simulink library "xps_library"  (Simulink 8.2)
settings: Solver=ode45  SolverMode=SingleTasking  StartTime=0.0  StopTime=10.0  RelTol=1e-3
undefined symbols (not defined in the file): sys_clk
libraries: xbsIndex_r4 x865, dspsigops x81, simulink x68, casper_library_flow_control x68, xps_library x25, casper_library_misc x4
(part 1 of 10)
settings Model: ForwardingTableString=||__slOldName__||xps_library/XSG core config||__slNewName__||xps_library/XSG_core_config||__slTransformationFcn__||XSG core config||__slOldName__||xps_library/Shared BRAM||__slNewName__||xps_library/Shared_BRAM||__slTransformationFcn__||Shared BRAM||__slOldName__||xps_library/software register||__slNewName__||xps_library/software_register||__slTransformationFcn__||Software Regsiter  Creator=hchen05  LastModifiedBy=jackh

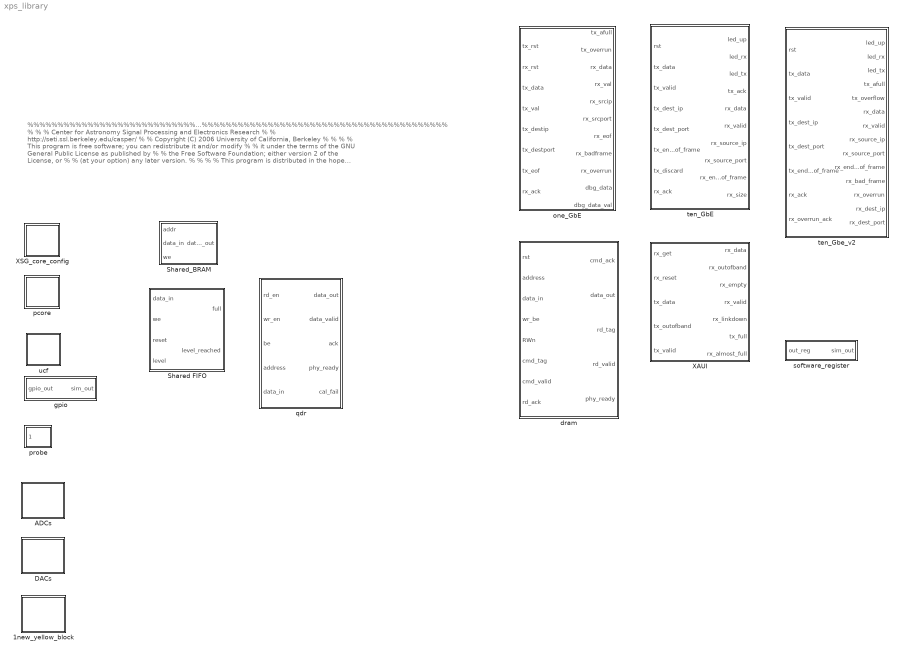
== system xps_library ==
  note: %%%%%%%%%%%%%%%%%%%%%%%%%%%%%%%%%%%%%%%%%%%%%%%%%%%%%%%%%%%%%%%%%%%%%%%%%%%%%%%
      | %                                                                             %
      | %   Center for Astronomy Signal Processing and Electronics Research           %
      | %   http://seti.ssl.berkeley.edu/casper/                                      %
      | %   Copyright (C) 2006 University of California, Berkeley                     %
      | %                                                                             %
      | %   This program is free software; you can redistribute it and/or modify      %
      | %   it under the terms of the GNU General Public License as published by      %
      | %   the Free Software Foundation; either version 2 of the License, or         %
      | %   (at your option) any later version.                                       %
      | %                                                                             %
      | %   This program is distributed in the hope that it will be useful,           %
      | %   but WITHOUT ANY WARRANTY; without even the implied warranty of            %
      | %   MERCHANTABILITY or FITNESS FOR A PARTICULAR PURPOSE.  See the             %
      | %   GNU General Public License for more details.                              %
      | %                                                                             %
      | %   You should have received a copy of the GNU General Public License along   %
      | %   with this program; if not, write to the Free Software Foundation, Inc.,   %
      | %   51 Franklin Street, Fifth Floor, Boston, MA 02110-1301 USA.               %
      | %                                                                             %
      | %%%%%%%%%%%%%%%%%%%%%%%%%%%%%%%%%%%%%%%%%%%%%%%%%%%%%%%%%%%%%%%%%%%%%%%%%%%%%%%
  1new_yellow_block : Subsystem  Tag=xps:block_name
  ADCs : Subsystem
  DACs : Subsystem
  Shared FIFO : Subsystem  Tag=xps:fifo  mask{io_dir=To Processor, arith_type=Unsigned, data_width=32, data_bin_pt=0, fifo_length=512}
      mask prompts: io_dir "I/O Direction:"; arith_type "Data Type:"; data_width "Data Width:"; data_bin_pt "Data Binary Point:"; fifo_length "Depth:"
      mask init:
      | fifo_mask;
      mask TypeOptions io_dir: From Processor | To Processor
      mask TypeOptions arith_type: Unsigned | Signed  (2's comp)
      mask TypeOptions data_width: 4 | 8 | 16 | 32 | 64 | 128 | 256
      mask TypeOptions fifo_length: 512 | 1024 | 2048 | 4096 | 8192 | 16384 | 32768 | 65536
  Shared_BRAM : Subsystem  Tag=xps:bram  mask{arith_type=Unsigned, addr_width=10, data_width=32, reg_prim_output=off, reg_core_output=off, optimization=Minimum_Area, data_bin_pt=0, init_vals=[0:2^10-1], sample_rate=1}
      mask prompts: arith_type "Output Data Type"; addr_width "Address width"; data_width "Data Width"; reg_prim_output "Register Primitive Output"; reg_core_output "Register Core Output"; data_bin_pt "Data Binary Point"; init_vals "Initial values (simulation only)"; sample_rate "Sample rate"
      mask init:
      | shared_bram_mask;
      mask TypeOptions arith_type: Unsigned | Signed  (2's comp)
      mask TypeOptions data_width: 8 | 16 | 32 | 64 | 128
      mask TypeOptions optimization: Minimum_Area | Low_Power
  XAUI : Subsystem  Tag=xps:xaui  mask(xaui){demux=1, port=ROACH:0, open_phy=on, show_param=off, pre_emph=3, swing=800}
      mask prompts: open_phy "Use KAT open PHY"; show_param "---------------------- Show Implementation Parameters -----------------------------------------------------------------------------------"; pre_emph "Pre-emphasis"; swing "Differential swing"
      mask help: XAUI block for sending and receiving point-to-point, streaming data over the ROACH1 CX4 connectors. NOTE: A new version of this block is in development.
      mask init:
      | xaui_mask;
      mask Help: eval('xlWeb([getenv(''MLIB_ROOT''), ''\doc\html\com_xaui\com_xaui.html''])')
      mask TypeOptions demux: 1 | 2
      mask TypeOptions port: ROACH:0 | ROACH:1 | ROACH:2 | ROACH:3
      mask Callback show_param:
      | myname=gcb;
      | if strcmp(get_param(myname, 'show_param'), 'on')
      |     set_param(myname, 'MaskVisibilities', {'on','on','on','on','on','on'});
      | else
      |     set_param(myname, 'MaskVisibilities', {'on','on','on','on','off','off'});
      | end
      mask TypeOptions pre_emph: 0 | 1 | 2 | 3
      mask TypeOptions swing: 400 | 500 | 600 | 700 | 800
  XSG_core_config : Subsystem  Tag=xps:xsg  mask(xsg core config){hw_sys=ROACH2:sx475t, clk_src=sys_clk, ROACH_clk_src=sys_clk, ROACH2_clk_src=sys_clk, MKDIG_clk_src=sys_clk, clk_rate=100, sample_period=1, synthesis_tool=XST}
      mask prompts: hw_sys "Hardware Platform"; clk_src "User IP Clock source"; ROACH_clk_src "User IP Clock Source"; ROACH2_clk_src "User IP Clock Source"; MKDIG_clk_src "User IP Clock Source"; clk_rate "User IP Clock Rate (MHz)"; sample_period "Sample Period"; synthesis_tool "Synthesis Tool:"
      mask help:
      | The XSG Core Config block is used to configure the System Generator design
      | for the casper_xps toolflow. Settings here are used to configure the
      | Xilinx System Generator block parameters automatically, and control toolflow
      | script  execution. It needs to be at the top level of all designs being compiled
      | with the casper_xps toolflow.
      mask init:
      | xps_xsg_conf_mask;
      mask Help: eval('xlWeb([getenv(''MLIB_ROOT''), ''\doc\html\sys_xsg_core_config\sys_xsg_core_config.html''])')
      mask TypeOptions hw_sys: ROACH:sx95t | ROACH:lx110t | ROACH2:sx475t | MKDIG
      mask Callback hw_sys: xps_xsg_conf_callback;
      mask TypeOptions ROACH_clk_src: sys_clk | sys_clk2x | arb_clk | aux0_clk | aux0_clk2x | aux1_clk | aux1_clk2x | adc0_clk | adc1_clk | dac0_clk | dac1_clk
      mask Callback ROACH_clk_src: xps_xsg_conf_callback;
      mask TypeOptions ROACH2_clk_src: sys_clk | aux_clk | adc0_clk | adc1_clk | dac0_clk | dac1_clk
      mask Callback ROACH2_clk_src: xps_xsg_conf_callback;
      mask TypeOptions MKDIG_clk_src: sys_clk | adc_clk
      mask Callback MKDIG_clk_src: xps_xsg_conf_callback;
      mask TypeOptions synthesis_tool: Leonardo Spectrum | Synplify | Synplify Pro | XST
      mask Display: fprintf(['MSSGE\n', hw_sys]);
  dram : Subsystem  Tag=xps:dram  mask(dram){dimm=1, arith_type=Unsigned, bin_pt=0, ip_clock=200, sample_period=1, bram_fifos=on, disable_tag=on, ram_depth=18, bank_mgt=off, wide_data=off, half_burst=off, use_sniffer=on}
      mask prompts: arith_type "Data Type"; bin_pt "Data binary point"; ip_clock "Datapath clock rate (MHz)"; sample_period "Sample period"; bram_fifos "Use BRAM FIFOs"; disable_tag "Disable tag FIFO"; ram_depth "Simulation address width"; bank_mgt "Enable bank management"; wide_data "Use wide data bus (288 bits)"; half_burst "Use half-burst"; use_sniffer "Include CPU Interface"
      mask help:
      | Interface to 1GB DDR2 DIMM of ROACH1 and the 2-4GB DDR3 DIMM of ROACH2.
      | Commands that are clocked-in are executed with an unknown delay, however, execution order is maintained.
      mask init:
      | dram_mask(gcb, wide_data);
      mask TypeOptions dimm: 1
      mask TypeOptions arith_type: Boolean | Unsigned | Signed  (2's comp)
      mask Callback wide_data:
      | myname=gcb;
      | if strcmp(get_param(myname, 'wide_data'), 'off')
      |     masks = get_param(myname, 'MaskEnables');
      |     masks{12} = 'on';
      |     set_param(myname, 'MaskEnables', masks);
      | else
      |     set_param(myname, 'half_burst', 'off');
      |     masks = get_param(myname, 'MaskEnables');
      |     masks{12} = 'off';
      |     set_param(myname, 'MaskEnables', masks);
      | end
  gpio : Subsystem  Tag=xps:gpio  mask(gpio){io_group=ROACH:aux0_clk, io_dir=out, arith_type=Boolean, bitwidth=1, bin_pt=0, bit_index=0, sample_period=1, use_single_ended=off, use_ddr=off, reg_iob=on, reg_clk_phase=0, termination=None}
      mask prompts: io_group "I/O group"; io_dir "I/O direction"; arith_type "Data Type"; bitwidth "Data bitwidth"; bin_pt "Data binary point"; bit_index "GPIO bit index"; sample_period "Sample period"; use_single_ended "Use as single-ended"; use_ddr "Use DDR"; reg_iob "Pack register in the pad"; reg_clk_phase "Register clock phase"; termination "Termination method"
      mask help: GPIO interfaces for ROACH and ROACH2 boards.
      mask init:
      | gpio_mask;
      mask TypeOptions io_group: ROACH:aux0_clk | ROACH:aux1_clk | ROACH:led | ROACH:gpioa | ROACH:gpioa_oe_n | ROACH:gpiob | ROACH:gpiob_oe_n | ROACH:qsh | ROACH:zdok0 | ROACH:zdok1 | ROACH2:aux_clk | ROACH2:led | ROACH2:gpio | ROACH2:qsh | ROACH2:sync_in | ROACH2:sync_out | ROACH2:zdok0 | ROACH2:zdok1
      mask Callback io_group:
      | if ~isempty(find(strcmp(get_param(gcb, 'io_group'), {'ROACH:qsh' 'ROACH:zdok0' 'ROACH:zdok1' 'ROACH2:sync_in' 'ROACH2:sync_out'})))
      |     set_param(gcb, 'MaskVisibilities', {'on','on','on','on','on','on','on','on','on','on','on','on'});
      | else
      |     set_param(gcb, 'MaskVisibilities', {'on','on','on','on','on','on','on','off','on','on','on','on'});
      | end
      mask TypeOptions io_dir: in | out
      mask Callback io_dir:
      | if ~isempty(find(strcmp(get_param(gcb, 'io_group'), {'ROACH:qsh' 'ROACH:zdok0' 'ROACH:zdok1' 'ROACH2:sync_in' 'ROACH2:sync_out'})))
      |     set_param(gcb, 'MaskVisibilities', {'on','on','on','on','on','on','on','on','on','on','on','on'});
      | else
      |     set_param(gcb, 'MaskVisibilities', {'on','on','on','on','on','on','on','off','on','on','on','on'});
      | end
      mask TypeOptions arith_type: Boolean | Unsigned | Signed  (2's comp)
      mask Callback use_ddr:
      | if strcmp(get_param(gcb,'use_ddr'),'on')
      |     set_param(gcb,'reg_iob','on');
      |     set_param(gcb,'MaskEnables', {'on' 'on' 'on' 'on' 'on' 'on' 'on' 'on' 'on' 'off' 'on' 'on'});
      | else
      |     set_param(gcb,'MaskEnables', {'on' 'on' 'on' 'on' 'on' 'on' 'on' 'on' 'on' 'on' 'on' 'on'});
      | end
      mask TypeOptions reg_clk_phase: 0 | 90 | 180 | 270
      mask TypeOptions termination: None | Pullup | Pulldown
  one_GbE : Subsystem  Tag=xps:onegbe  mask(one_GbE){local_en=on, dis_cpu_rx=off, dis_cpu_tx=off, cpu_promiscuous=on, local_mac=hex2dec('123456789abc'), local_ip=hex2dec('c0a8290a'), local_port=4321, local_gateway=1}
      mask prompts: local_en "Enable fabric on startup"; dis_cpu_rx "Disable CPU Rx"; dis_cpu_tx "Disable CPU Tx"; cpu_promiscuous "CPU Promiscuous"; local_mac "Fabric MAC Address"; local_ip "Fabric IP Address"; local_port "Fabric UDP Port"; local_gateway "Fabric Gateway"
      mask help: This block sends and receives UDP frames (packets). It accepts a 8 bit wide data stream with user-determined frame breaks. The data stream is wrapped in a UDP frame for transmission. Incoming UDP packets are unwrapped and the data presented as a 8 bit wide stream.
      mask init:
      | onegbe_mask;
      mask Help: eval('xlWeb([getenv(''MLIB_ROOT''), ''\doc\html\com_ten_GbE\com_ten_GbE.html''])')
  pcore : Subsystem  Tag=xps:pcore  mask(pcore){pcore_path=customlib/pcores}
      mask prompts: pcore_path "Custom pcores path"
      mask help: Allows insertion of custom EDK pcores not distributed with base systems.
      mask Display: fprintf('PCORE');
  probe : Subsystem  Tag=xps:probe  mask{ila_number=0, match_type=basic, match_counter_width=8, capture_depth=512, arith_type=Boolean, bitwidth=1, bin_pt=0}
      mask prompts: ila_number "Chipscope ILA number"; match_type "Match Unit Type"; match_counter_width "Match counter width"; capture_depth "Probe capture depth"; arith_type "Data type"; bitwidth "Data bit width"; bin_pt "Data binary point"
      mask init:
      | probe_mask;
      mask TypeOptions ila_number: 0 | 1 | 2 | 3 | 4 | 5 | 6 | 7 | 8 | 9 | 10 | 11 | 12 | 13 | 14
      mask TypeOptions match_type: basic | basic with edges | extended | extended with edges | range | range with edges
      mask TypeOptions match_counter_width: 0 | 8 | 16 | 24 | 32
      mask TypeOptions capture_depth: 512 | 1024 | 2048 | 4096 | 8192 | 16384
      mask TypeOptions arith_type: Boolean | Unsigned | Signed  (2's comp)
  qdr : Subsystem  Tag=xps:qdr  mask(qdr){which_qdr=qdr0, qdr_awidth=12, use_sniffer=on}
      mask prompts: which_qdr "QDR Chip"; qdr_awidth "Simulation QDR address width"; use_sniffer "Include CPU Interface"
      mask help:
      | Interface to the QDR II SRAM device on ROACH and ROACH2.
      | For ROACH, use only QDR chips qdr0 or qdr1.
      | For ROACH2, use qdr chips qdr0, qdr1, qdr2 or qdr3.
      mask init:
      | qdr_mask(gcb);
      mask TypeOptions which_qdr: qdr0 | qdr1 | qdr2 | qdr3
  software_register : Subsystem  Tag=xps:sw_reg  mask(swreg){io_dir=To Processor, io_delay=0, sample_period=1, names=reg, bitwidths=32, bin_pts=0, arith_types=0, sim_port=on, show_format=on}
      mask prompts: io_dir "I/O direction"; io_delay "I/O delay"; sample_period "Sample period"; names "Bitfield names [msb...lsb]"; bitwidths "Bitfield widths"; bin_pts "Bitfield binary pts"; arith_types "Bitfield types, ufix=0, fix=1, bool=2"; sim_port "Provide sim input/output?"; show_format "Print format string?"
      mask help: A 32-bit software-accessible register. Can be divided into bitfields of varying widths and types using the fields in the block mask.
      mask init:
      | try
      |     swreg_init(gcb)
      | catch ex
      |     disp(sprintf('%s: %s', gcb, ex.message))
      |     errordlg(ex.message)
      | end
      settings: AttributesFormatString=1output:uf32.0 = 32 bits
      mask TypeOptions io_dir: To Processor | From Processor
      mask Callback io_dir:
      | mask_enables = get_param(gcb, 'MaskEnables');
      | mask_names = get_param(gcb, 'MaskNames');
      | if strcmp(get_param(gcb, 'io_dir'), 'To Processor'),
      |     mask_enables{ismember(mask_names, 'sample_period')} = 'off';
      | else
      |     mask_enables{ismember(mask_names, 'sample_period')} = 'on';
      | end
      | set_param(gcb, 'MaskEnables', mask_enables);
  ten_GbE : Subsystem  Tag=xps:tengbe  mask(ten_GbE){port=ROACH:0, mac_lite=off, open_phy=off, show_param=off, pre_emph=3, swing=800, fab_en=off, fab_mac=0, fab_ip=0, fab_udp=0, fab_gate=0}
      mask prompts: mac_lite "Use light-weight MAC: Warning --> it DOES NOT check any CRC on receive"; open_phy "Use KAT open XAUI PHY"; show_param "---------------------- Show Implementation Parameters -----------------------------------------------------------------------------------"; pre_emph "Pre-emphasis"; swing "Differential swing"; fab_en "Enable fabric on startup"; fab_mac "Fabric MAC Address"; fab_ip "Fabric IP Address"; fab_udp "Fabric UDP Port"; fab_gate "Fabric Gateway"
      mask help: This block sends and receives UDP frames (packets). It accepts a 64 bit wide data stream with user-determined frame breaks. The data stream is wrapped in a UDP frame for transmission. Incoming UDP packets are unwrapped and the data presented as a 64 bit wide stream.
      mask init:
      | tengbe_mask;
      mask Help: eval('xlWeb([getenv(''MLIB_ROOT''), ''\doc\html\com_ten_GbE\com_ten_GbE.html''])')
      mask TypeOptions port: ROACH:0 | ROACH:1 | ROACH:2 | ROACH:3
      mask Callback show_param:
      | myname=gcb;
      | if strcmp(get_param(myname, 'show_param'), 'on')
      |     set_param(myname, 'MaskVisibilities', {'on','on','on','on','on', 'on','on','on','on','on', 'on',});
      | else
      |     set_param(myname, 'MaskVisibilities', {'on','on','on','on','off','off','off','off','off','off','off'});
      | end
      mask TypeOptions pre_emph: 0 | 1 | 2 | 3
      mask TypeOptions swing: 400 | 500 | 600 | 700 | 800
  ten_Gbe_v2 : Subsystem  Tag=xps:tengbe_v2  mask(ten_GbE_v2){flavour=sfp+, slot=0, port_r1=0, port_r2_cx4=0, port_r2_sfpp=0, rx_dist_ram=off, large_frames=off, show_param=off, pre_emph_r2=1.07, pre_emph=3, post_emph_r2=0.18, rxeqmix_r2=7, swing_r2=940, swing=800, fab_en=on, fab_mac=hex2dec('123456780000'), fab_ip=192*(2^24) + 168*(2^16) + 5*(2^8) + 20*(2^0), fab_udp=10000, fab_gate=1, cpu_rx_en=on, cpu_tx_en=on, ttl=hex2dec('FF'), promisc_mode=off, debug_ctr_width=16, txctr=off, txerrctr=off, txerrctr_len=100, txofctr=off, txfullctr=off, txvldctr=off, txsnaplen=0 - no snap, rxctr=off, rxerrctr=off, rxerrctr_len=100, rxofctr=off, rxbadctr=off, rxvldctr=off, rxeofctr=off, rxsnaplen=0 - no snap}
      mask prompts: flavour "Mezzanine card flavour"; slot "Card slot"; port_r1 "Port"; port_r2_cx4 "Port"; port_r2_sfpp "Port"; rx_dist_ram "Shallow RX Fifo (Beware overruns!)"; large_frames "Enable Large TX Frames (8k+512)"; show_param "---------------------- Show Implementation Parameters -----------------------------------------------------------------------------------"; pre_emph_r2 "Pre-emphasis (dB)"; pre_emph "Pre-emphasis"; post_emph_r2 "Post-emphasis (dB)"; rxeqmix_r2 "Receive equalisation"; swing_r2 "Driver Swing Control (mVppd)"; swing "Differential swing"; fab_en "Enable fabric on startup"; fab_mac "Fabric MAC Address"; fab_ip "Fabric IP Address"; fab_udp "Fabric UDP Port"; fab_gate "Fabric Gateway"; cpu_rx_en "Enable CPU RX"; cpu_tx_en "Enable CPU TX"; promisc_mode "Promiscuous mode"; debug_ctr_width "Debug counter width"; txctr "TX - core_txctr"; txerrctr "TX packet length error - core_txerrctr"; txerrctr_len "-- expected TX packet length"; txofctr "TX overflow - core_txofctr"; txfullctr "TX full - core_txfullctr"; txvldctr "TX valid cycle - core_txvldctr"; txsnaplen "TX snapshot length"; rxctr "RX - core_rxctr"; rxerrctr "RX packet length error - core_rxerrctr"; rxerrctr_len "-- expected RX packet length"; rxofctr "RX overflow - core_rxofctr"; rxbadctr "RX bad - core_rxbadctr"; rxvldctr "RX valid cycle - core_rxvldctr"; rxeofctr "RX eof - core_rxeofctr"; rxsnaplen "RX snapshot length"
      mask help: This block sends and receives UDP frames (packets). It accepts a 64 bit wide data stream with user-determined frame breaks. The data stream is wrapped in a UDP frame for transmission. Incoming UDP packets are unwrapped and the data presented as a 64 bit wide stream.
      mask init:
      | temp = eval(get_param(gcb, 'debug_ctr_width'));
      | if temp <= 0,
      |     error('Debug counters cannot be ltoet zero.');
      | end
      | tengbe_v2_mask(gcb)
      mask TypeOptions flavour: sfp+ | cx4
      mask Callback flavour: tengbe_v2_callback
      mask TypeOptions slot: 0 | 1
      mask TypeOptions port_r1: 0 | 1 | 2 | 3
      mask TypeOptions port_r2_cx4: 0 | 1 | 2
      mask TypeOptions port_r2_sfpp: 0 | 1 | 2 | 3
      mask Callback show_param: tengbe_v2_callback
      mask TypeOptions pre_emph_r2: 0.15 | 0.3 | 0.45 | 0.61 | 0.74 | 0.91 | 1.07 | 1.25 | 1.36 | 1.55 | 1.74 | 1.94 | 2.11 | 2.32 | 2.54 | 2.77
      mask TypeOptions pre_emph: 0 | 1 | 2 | 3
      mask TypeOptions post_emph_r2: 0.18 | 0.19 | 0.2 | 0.39 | 0.63 | 0.82 | 1.07 | 1.32 | 1.6 | 1.65 | 1.94 | 2.21 | 2.52 | 2.76 | 3.08 | 3.41 | 3.77 | 3.97 | 4.36 | 4.73 | 5.16 | 5.47 | 5.93 | 6.38 | 6.89
      mask TypeOptions rxeqmix_r2: 0 | 1 | 2 | 3 | 4 | 5 | 6 | 7
      mask TypeOptions swing_r2: 110 | 210 | 310 | 400 | 480 | 570 | 660 | 740 | 810 | 880 | 940 | 990 | 1040 | 1080 | 1110 | 1130
      mask TypeOptions swing: 400 | 500 | 600 | 700 | 800
      mask Callback txerrctr:
      | blk = gcb;
      | mask_visibilities = get_param(blk, 'MaskVisibilities');
      | mask_names = get_param(blk, 'MaskNames');
      | if strcmp(get_param(blk, 'txerrctr'), 'on')
      |     mask_visibilities{ismember(mask_names, 'txerrctr_len')} = 'on';
      | else
      |     mask_visibilities{ismember(mask_names, 'txerrctr_len')} = 'off';
      | end
      | set_param(blk, 'MaskVisibilities', mask_visibilities);
      mask TypeOptions txsnaplen: 0 - no snap | 256 | 512 | 1024 | 2048 | 4096 | 8192 | 16384
      mask Callback rxerrctr:
      | blk = gcb;
      | mask_visibilities = get_param(blk, 'MaskVisibilities');
      | mask_names = get_param(blk, 'MaskNames');
      | if strcmp(get_param(blk, 'rxerrctr'), 'on')
      |     mask_visibilities{ismember(mask_names, 'rxerrctr_len')} = 'on';
      | else
      |     mask_visibilities{ismember(mask_names, 'rxerrctr_len')} = 'off';
      | end
      | set_param(blk, 'MaskVisibilities', mask_visibilities);
      mask TypeOptions rxsnaplen: 0 - no snap | 256 | 512 | 1024 | 2048 | 4096 | 8192 | 16384
  ucf : Subsystem  Tag=xps:ucf  mask(ucf){ucf_file=/tmp/testucf.ucf}
      mask prompts: ucf_file "Path to file containing constraints. (This should adhere to .ucf syntax)"
      mask help: Allows insertion of custom constraints into a compile.
      mask Display: fprintf('UCF');

== system xps_library/1new_yellow_block ==

== system xps_library/ADCs ==
  adc : Subsystem  Tag=xps:adc  mask(adc){adc_brd=adc0, adc_clk_rate=800, adc_interleave=on, sample_period=1}
      mask prompts: adc_brd "ADC board"; adc_clk_rate "ADC clock rate (MHz)"; adc_interleave "ADC interleave mode"; sample_period "Sample period"
      mask help: The ADC block converts analog inputs to digital outputs. Every clock cycle, the inputs are sampled and digitized to 8 bit binary point numbers in the range of [-1, 1) and are then output by the adc.
      mask init:
      | adc_mask;
      mask Help: eval('xlWeb([getenv(''MLIB_ROOT''), ''\doc\html\sys_adc\sys_adc.html''])')
      mask TypeOptions adc_brd: adc0 | adc1
  adc083000_ctrl : Subsystem  Tag=xps:adc083000_ctrl  mask(adc083000_ctrl){}
      mask init:
      | adc083000_ctrl_mask;
  adc083000x2 : Subsystem  Tag=xps:adc083000x2  mask(adc_083000x2){use_adc0=on, use_adc1=on, demux_adc=off, clock_sync=on, verbose=off, using_ctrl=on, adc_clk_rate=1000, sample_period=1, bit_width=8}
      mask prompts: use_adc0 "Use ZD0K0?"; use_adc1 "Use ZDOK1?"; demux_adc "Demux ADCs by 2?"; clock_sync "Interleave 2 ADC boards?"; verbose "Verbose Block Creation?"; using_ctrl "Add ports for control registers?"; adc_clk_rate "ADC clock rate (MHz)"; sample_period "Sample Period"; bit_width "Output Bit Width"
      mask help:
      | The ADC block converts analog inputs to digital outputs.
      | Every clock cycle, the inputs are sampled and digitized to
      | 8 bit binary point numbers in the range of [-1, 1).
      |
      | Online block-specific documentation: http://casper.berkeley.edu/wiki/Adc083000
      mask init:
      | adc083000_mask;
      mask Help: eval('xlWeb([getenv(''MLIB_ROOT''), ''\doc\html\sys_adc\sys_adc.html''])')
  adc16x250-8 : Subsystem  Tag=xps:adc16  mask(ADC16){board_count=1, roach2_rev=2, zdok_rev=2}
      mask prompts: board_count "Number of ADC16 Boards"; roach2_rev "ROACH2 Revision"; zdok_rev "ZDOK Pinout Revision"
      mask help: 16-input ADC. When using one ADC16 board, it must be in ZDOK0.
      mask init:
      | % Only board_count is needed by init function
      | adc16_init(gcb, ...
      |     'board_count', board_count);
      settings: AttributesFormatString=r2 rev%<roach2_rev>\nzdok rev%<zdok_rev>
      mask Help:
      | This is the CASPER "yellow block" for the CASPER ADC16 board.  Each ADC
      | board has four ADC chips.  Each ADC chip accepts four inputs.  The four
      | 8-bit outputs from each ADC chip are concatenated into a 32-bit signal.
      mask TypeOptions board_count: 1 | 2
      mask TypeOptions roach2_rev: 1 | 2
      mask TypeOptions zdok_rev: 1 | 2
  adc1x1800-10 : Subsystem  Tag=xps:mkadc  mask(mkadc){adc_brd=adc0, adc_clk_rate=1800, sample_period=1, gray_en=on}
      mask prompts: adc_brd "ADC board"; adc_clk_rate "ADC clock rate (MHz)"; sample_period "Sample period"; gray_en "Gray Code Enable"
      mask help:
      | ADC1x1800-10
      | Single Input, Max 1.8G Sample, 10bit
      | Demux by 4
      | ADC: e2v AT84AS008CGL
      | DEMUX by 2: AT84CS001VTP
      | DEMUX by 2: FPGA
      mask init:
      | mkadc_mask;
      mask Help: ADC1x1800
      mask TypeOptions adc_brd: adc0 | adc1
  adc2x14_400 : Subsystem  Tag=xps:adc2x14_400  mask(ADC board 2xADS5474 Interface Block){adc_brd=0, adc_clk_rate=400}
      mask prompts: adc_brd "ADC Board"; adc_clk_rate "ADC Clock Rate (MHz)"
      mask help: Interface block for the MKID 14-bits 400 MHz ADC board (2xADS5474).
      mask init:
      | adc2x14_400_mask;
      mask TypeOptions adc_brd: 0 | 1
  adc2x14_400_4x : Subsystem  Tag=xps:adc2x14_400_4x  mask(2x 14-400 ADC Interface Block){adc_brd=1, adc_clk_rate=400}
      mask prompts: adc_brd "ADC Board"; adc_clk_rate "ADC Clock Rate (MHz)"
      mask help: Interface block for the 14-bits 400 MHz DC board (2xADS5474).
      mask init:
      | adc2x14_400_4x_mask;
      mask TypeOptions adc_brd: 0 | 1
  adc_mkid : Subsystem  Tag=xps:adc_mkid  mask(MKID ADC Interface Block){adc_brd=1, adc_clk_rate=512}
      mask prompts: adc_brd "ADC Board"; adc_clk_rate "ADC Clock Rate (MHz)"
      mask help: Interface block for the MKID 12-bits 550 MHz ADC board (2xADS54RF63).
      mask init:
      | adc_mkid_mask;
      mask TypeOptions adc_brd: 0 | 1
  adc_mkid_4x : Subsystem  Tag=xps:adc_mkid_4x  mask(MKID ADC Interface Block){adc_brd=1, adc_clk_rate=540}
      mask prompts: adc_brd "ADC Board"; adc_clk_rate "ADC Clock Rate (MHz)"
      mask help: Interface block for the MKID 12-bits ADC board (2xADS54RF63).
      mask init:
      | adc_mkid_4x_mask;
      mask TypeOptions adc_brd: 0 | 1
  adc_sim : Subsystem  mask(adc_sim){nStreams=8, bit_width=8}
      mask prompts: nStreams "Number of Output Streams"; bit_width "Sample Bit Width"
      mask help:
      | This block simulates the behavior of a demuxed ADC, which takes
      | as input a waveform and returns digital samples in parallel at
      | a slower rate.
      |
      | This block is used to simulate the behavior
      mask init:
      | adc_sim_init(gcb, ...
      |     'nStreams', nStreams, ...
      |     'bit_width', bit_width);
  asiaa_adc5g : Subsystem  Tag=xps:adc5g  mask(adc5g){input_mode=One-channel -- A, adc_brd=ZDOK 0, demux=1:2, adc_bit_width=4, adc_clk_rate=2500, using_ctrl=on, test_ramp=off}
      mask prompts: input_mode "Input mode:"; adc_brd "ADC Board"; demux "Internal demux"; adc_bit_width "ADC Resolution (bits):"; adc_clk_rate "ADC Clock Rate (MHz):"; using_ctrl "use control"; test_ramp "start in test ramp mode"
      mask help:
      | Interface for the ASIAA 5 GSps ADC. Supports interleaving all four
      | cores using either input A or C, or interleaving two-cores each for
      | A and C. The hardware itself comes in two versions:
      |
      | DMUX 1:2 -- 4-bit samples, 4 parallel streams
      | DMUX 1:1 -- 8-bit samples, 2 parallel streams
      |
      | In either configuration this block will output 8 parallel streams
      | but the underlying interface, and the bitwidth of the samples,
      | will be different.
      mask init:
      | adc5g_init(gcb,...
      |     'input_mode', input_mode,...
      |     'demux', demux,...
      |     'adc_clk_rate', adc_clk_rate,...
      |     'adc_bit_width', adc_bit_width,...
      |     'adc_brd', adc_brd,...
      |     'using_ctrl', using_ctrl,...
      |     'test_ramp', test_ramp);
      mask TypeOptions input_mode: One-channel -- A | One-channel -- C | Two-channel -- A&C
      mask TypeOptions adc_brd: ZDOK 0 | ZDOK 1
      mask TypeOptions demux: 1:1 | 1:2
      mask Callback demux:
      | demux = get_param(gcb,'demux');
      | if(strcmp(demux,'1:1')),
      |     set_param(gcb, 'adc_bit_width', '8')
      | elseif(strcmp(demux, '1:2')),
      |     set_param(gcb, 'adc_bit_width', '4');
      | else
      | end
  conv : Subsystem  mask{bit_width=8}
      mask prompts: bit_width "Bit Width"
      mask help:
      | Converts an (8-bit) unsigned number to 2's complement.
      | This block should eventually be able to handle arbitrary
      | width inputs.
      mask init:
      | % set_param([gcb, '/Slice1'], 'nbits', num2str(bit_width-1));
      | % set_param([gcb, '/Reinterpret'], 'bin_pt', num2str(bit_width-1));
  generic_adc : Subsystem  mask(generic_adc){in=1, out=4, bits=8, interleaved=off, or_support=off, sync_support=on, dv_support=off}
      mask prompts: in "inputs"; out "outputs per input"; bits "adc bit width"; interleaved "interleaved mode"; or_support "over-range support"; sync_support "sync support"; dv_support "data valid support"
      mask help: Generic ADC simulation block
      mask init:
      | generic_adc_init(gcb, ...
      |     'in', in, ...
      |     'out', out, ...
      |     'bits', bits, ...    
      |     'interleaved', interleaved, ...
      |     'or_support', or_support, ...
      |     'sync_support', sync_support, ...
      |     'dv_support', dv_support);
  katadc : Subsystem  Tag=xps:katadc  mask(katadc){adc_brd=adc0, adc_interleave=off, bypass_auto=off, en_gain=on, adc_clk_rate=800, sample_period=1}
      mask prompts: adc_brd "ADC board"; adc_interleave "ADC interleave mode"; bypass_auto "Bypass auto config"; en_gain "Enable gain"; adc_clk_rate "ADC sampling rate (MHz)"; sample_period "Sample period"
      mask init:
      | name = gcb;
      | katadc_init(gcb, ...
      |     'name', name, ...
      |     'adc_brd', adc_brd, ...
      |     'adc_interleave', adc_interleave, ...
      |     'bypass_auto', bypass_auto, ...
      |     'en_gain', en_gain, ...
      |     'adc_clk_rate', adc_clk_rate, ...
      |     'sample_period', sample_period);
      mask TypeOptions adc_brd: adc0 | adc1
  of1 : Subsystem  mask(of){bit_num=0, n_adc_bits=8}
      mask prompts: bit_num "Bit index of overflow detection bus:"; n_adc_bits "Number of bits in ADC"
      mask help: 1-cycle overflow detector for an n-bit ADC outputs (simulation only)
  of_detect_bus : Subsystem  mask(of_detect_bus){nStreams=8, bit_width=8}
      mask prompts: nStreams "Number of Streams"; bit_width "Bit Width"
      mask init:
      | of_detect_bus_init(gcb, ...
      |     'nStreams', nStreams, ...
      |     'bit_width', bit_width);
  quadc : Subsystem  Tag=xps:quadc  mask(CASPER QuADC Interface Block){adc_brd=0, adc_clk_rate=200}
      mask prompts: adc_brd "ADC Board"; adc_clk_rate "ADC Clock Rate (MHz)"
      mask help: Interface block for the CASPER Quad ADC board (ADC4x250-8).
      mask init:
      | quadc_mask;
      mask TypeOptions adc_brd: 0 | 1
  x64_adc : Subsystem  Tag=xps:x64_adc  mask(x64_adc){adc_clk_rate=12, spi=off, ctrl_gpio=GPIO_A}
      mask prompts: adc_clk_rate "ADC clock rate (MHz)"; spi "Include SPI interface?"; ctrl_gpio "GPIO bank to use for control signals?"
      mask help: The ADC block converts analog inputs to digital outputs. Every clock cycle, the inputs are sampled and digitized to 8 bit binary point numbers in the range of [-1, 1) and are then output by the adc.
      mask init:
      | x64_adc_mask(gcb, 'spi', spi);
      mask Help: eval('xlWeb([getenv(''MLIB_ROOT''), ''\doc\html\sys_adc\sys_adc.html''])')
      mask TypeOptions ctrl_gpio: GPIO_A | GPIO_B

== system xps_library/DACs ==
  dac_mkid : Subsystem  Tag=xps:dac_mkid  mask(MKID DAC Interface Block){dac_brd=0, dac_clk_rate=512, sample_period=1}
      mask prompts: dac_brd "DAC board"; dac_clk_rate "DAC external clock rate (MHz)"; sample_period "Sample period"
      mask help: Interface block for the MKID 16-bits DAC board (2xDAC5681)
      mask init:
      | dac_mkid_mask;
      mask TypeOptions dac_brd: 0 | 1
  dac_mkid_4x : Subsystem  Tag=xps:dac_mkid_4x  mask{dac_brd=0, dac_clk_rate=540, sample_period=1}
      mask prompts: dac_brd "DAC board"; dac_clk_rate "DAC external clock rate (MHz)"; sample_period "Sample period"
      mask init:
      | dac_mkid_4x_mask;
      mask TypeOptions dac_brd: 0 | 1

== system xps_library/Shared FIFO ==
  data_in : Inport
  we : Inport  Port=2
  reset : Inport  Port=3
  level : Inport  Port=4
  convert_untitled_Shared_FIFO_user_data_in : xbsIndex_r4/Convert  gui_display_data_type=Fixed-point  arith_type=Unsigned  n_bits=32  bin_pt=0  float_type=Single  exp_bits=8  fraction_bits=24  quantization=Truncate  overflow=Wrap  en=off  latency=0  dbl_ovrd=off  pipeline=off  block_type=convert
  convert_untitled_Shared_FIFO_user_level : xbsIndex_r4/Convert  gui_display_data_type=Fixed-point  arith_type=Unsigned  n_bits=16  bin_pt=0  float_type=Single  exp_bits=8  fraction_bits=24  quantization=Truncate  overflow=Wrap  en=off  latency=0  dbl_ovrd=off  pipeline=off  block_type=convert
  convert_untitled_Shared_FIFO_user_reset : xbsIndex_r4/Convert  gui_display_data_type=Fixed-point  arith_type=Unsigned  n_bits=1  bin_pt=0  float_type=Single  exp_bits=8  fraction_bits=24  quantization=Truncate  overflow=Wrap  en=off  latency=0  dbl_ovrd=off  pipeline=off  block_type=convert
  convert_untitled_Shared_FIFO_user_we : xbsIndex_r4/Convert  gui_display_data_type=Fixed-point  arith_type=Unsigned  n_bits=1  bin_pt=0  float_type=Single  exp_bits=8  fraction_bits=24  quantization=Truncate  overflow=Wrap  en=off  latency=0  dbl_ovrd=off  pipeline=off  block_type=convert
  untitled_Shared_FIFO_user_data_in : xbsIndex_r4/Gateway Out  hdl_port=on  timing_constraint=None  locs_specified=off  LOCs={}  block_type=gatewayout
      settings: infoedit="Gateway out block.  Converts Xilinx fixed point inputs into ouputs of type Simulink integer, double, or fixed point.<P><P>Hardware notes:  In hardware these blocks become top level output ports or are discarded, depending on how they are configured."
  untitled_Shared_FIFO_user_full : xbsIndex_r4/Gateway In  gui_display_data_type=Fixed-point  arith_type=Unsigned  n_bits=1  bin_pt=0  preci_type=Single  exp_width=8  frac_width=24  quantization="Round  (unbiased: +/- Inf)"  overflow=Saturate  period=1  dbl_ovrd=off  timing_constraint=None  locs_specified=off  LOCs={}  hdl_port=on  block_type=gatewayin
      settings: infoedit="Gateway in block.  Converts inputs of type Simulink integer, double and fixed point to  Xilinx fixed point type.<P><P>Hardware notes:  In hardware these blocks become top level input ports."
  untitled_Shared_FIFO_user_full_const : Constant  Value=0
  untitled_Shared_FIFO_user_level : xbsIndex_r4/Gateway Out  hdl_port=on  timing_constraint=None  locs_specified=off  LOCs={}  block_type=gatewayout
      settings: infoedit="Gateway out block.  Converts Xilinx fixed point inputs into ouputs of type Simulink integer, double, or fixed point.<P><P>Hardware notes:  In hardware these blocks become top level output ports or are discarded, depending on how they are configured."
  untitled_Shared_FIFO_user_level_reached : xbsIndex_r4/Gateway In  gui_display_data_type=Fixed-point  arith_type=Unsigned  n_bits=1  bin_pt=0  preci_type=Single  exp_width=8  frac_width=24  quantization="Round  (unbiased: +/- Inf)"  overflow=Saturate  period=1  dbl_ovrd=off  timing_constraint=None  locs_specified=off  LOCs={}  hdl_port=on  block_type=gatewayin
      settings: infoedit="Gateway in block.  Converts inputs of type Simulink integer, double and fixed point to  Xilinx fixed point type.<P><P>Hardware notes:  In hardware these blocks become top level input ports."
  untitled_Shared_FIFO_user_level_reached_const : Constant  Value=0
  untitled_Shared_FIFO_user_reset : xbsIndex_r4/Gateway Out  hdl_port=on  timing_constraint=None  locs_specified=off  LOCs={}  block_type=gatewayout
      settings: infoedit="Gateway out block.  Converts Xilinx fixed point inputs into ouputs of type Simulink integer, double, or fixed point.<P><P>Hardware notes:  In hardware these blocks become top level output ports or are discarded, depending on how they are configured."
  untitled_Shared_FIFO_user_we : xbsIndex_r4/Gateway Out  hdl_port=on  timing_constraint=None  locs_specified=off  LOCs={}  block_type=gatewayout
      settings: infoedit="Gateway out block.  Converts Xilinx fixed point inputs into ouputs of type Simulink integer, double, or fixed point.<P><P>Hardware notes:  In hardware these blocks become top level output ports or are discarded, depending on how they are configured."
  full : Outport
  level_reached : Outport  Port=2
  wires:
  untitled_Shared_FIFO_user_level_reached_const/1 -> untitled_Shared_FIFO_user_level_reached/1
  untitled_Shared_FIFO_user_level_reached/1 -> level_reached/1
  untitled_Shared_FIFO_user_full_const/1 -> untitled_Shared_FIFO_user_full/1
  untitled_Shared_FIFO_user_full/1 -> full/1
  convert_untitled_Shared_FIFO_user_level/1 -> untitled_Shared_FIFO_user_level/1
  level/1 -> convert_untitled_Shared_FIFO_user_level/1
  convert_untitled_Shared_FIFO_user_reset/1 -> untitled_Shared_FIFO_user_reset/1
  reset/1 -> convert_untitled_Shared_FIFO_user_reset/1
  convert_untitled_Shared_FIFO_user_we/1 -> untitled_Shared_FIFO_user_we/1
  we/1 -> convert_untitled_Shared_FIFO_user_we/1
  convert_untitled_Shared_FIFO_user_data_in/1 -> untitled_Shared_FIFO_user_data_in/1
  data_in/1 -> convert_untitled_Shared_FIFO_user_data_in/1

== system xps_library/Shared_BRAM ==
  addr : Inport
  data_in : Inport  Port=2
  we : Inport  Port=3
  calc_add : Subsystem  mask{data_width=32, addr_width=10, sample_rate=sample_rate}
      mask prompts: data_width "data width"; addr_width "address width"; sample_rate "sample rate"
  convert_addr : xbsIndex_r4/Convert  gui_display_data_type=Fixed-point  arith_type=Unsigned  n_bits=addr_width  bin_pt=0  float_type=Single  exp_bits=8  fraction_bits=24  quantization=Truncate  overflow=Wrap  en=off  latency=0  dbl_ovrd=off  pipeline=off  block_type=convert
      settings: xl_area=[0, 0, 0, 0, 0, 0, 0]
  convert_din1 : xbsIndex_r4/Convert  gui_display_data_type=Fixed-point  arith_type=Unsigned  n_bits=data_width  bin_pt=data_bin_pt  float_type=Single  exp_bits=8  fraction_bits=24  quantization=Truncate  overflow=Wrap  en=off  latency=0  dbl_ovrd=off  pipeline=off  block_type=convert
      settings: xl_area=[0, 0, 0, 0, 0, 0, 0]
  convert_we : xbsIndex_r4/Convert  gui_display_data_type=Fixed-point  arith_type=Unsigned  n_bits=1  bin_pt=0  float_type=Single  exp_bits=8  fraction_bits=24  quantization=Truncate  overflow=Wrap  en=off  latency=0  dbl_ovrd=off  pipeline=off  block_type=convert
      settings: xl_area=[0, 0, 0, 0, 0, 0, 0]
  mem : Subsystem
  munge_in : Subsystem  AncestorBlock=casper_library_flow_control/munge  mask(munge){divisions=1, div_size=32, order=[0], arith_type_out=Unsigned, bin_pt_out=0}
      mask prompts: divisions "Number of divisions"; div_size "Division size (bits)"; order "Division packing order"; arith_type_out "Output arithmetic type"; bin_pt_out "Output binary point"
      mask help: Splits an input bus into the specified number of divisions and then recombines them in the order specified (most significant division = 0,least = number divisions-1)
      mask init:
      | munge_init(gcb, ...
      |     'divisions', divisions, ...
      |     'div_size', div_size, ...
      |     'order', order, ...
      |     'arith_type_out', arith_type_out, ...
      |     'bin_pt_out', bin_pt_out);
      settings: AttributesFormatString=|
      | split:32
      | join:0
      | Unsigned [32,0]
      mask TypeOptions arith_type_out: Unsigned | Signed  (2's comp) | Floating-point
  munge_out : Subsystem  AncestorBlock=casper_library_flow_control/munge  mask(munge){divisions=1, div_size=32, order=[0], arith_type_out=Unsigned, bin_pt_out=0}
      mask prompts: divisions "Number of divisions"; div_size "Division size (bits)"; order "Division packing order"; arith_type_out "Output arithmetic type"; bin_pt_out "Output binary point"
      mask help: Splits an input bus into the specified number of divisions and then recombines them in the order specified (most significant division = 0,least = number divisions-1)
      mask init:
      | munge_init(gcb, ...
      |     'divisions', divisions, ...
      |     'div_size', div_size, ...
      |     'order', order, ...
      |     'arith_type_out', arith_type_out, ...
      |     'bin_pt_out', bin_pt_out);
      settings: AttributesFormatString=|
      | split:32
      | join:0
      | Unsigned [32,0]
      mask TypeOptions arith_type_out: Unsigned | Signed  (2's comp) | Floating-point
  untitled_Shared_BRAM_addr : xbsIndex_r4/Gateway Out  hdl_port=on  timing_constraint=None  locs_specified=off  LOCs={'A5','B9','A9','C1','A3','G6','E9','A6','A7','A8','B8','B1','B3','D9','B5','B4','B6','C2'}  block_type=gatewayout
      settings: infoedit="Gateway out block.  Converts Xilinx fixed point inputs into ouputs of type Simulink integer, double, or fixed point.<P><P>Hardware notes:  In hardware these blocks become top level output ports or are discarded, depending on how they are configured."  xl_area=[0, 0, 0, 0, 0, 0, 0]  sginterface={'Nallatech'=>{'xdspkit'=>{'non_memory_mapped_port'=>'uprev_Shared_BRAM_addr'}},'Xilinx'=>{'jtaghwcosim'=>{'non_memory_mapped_port'=>'uprev_Shared_BRAM_addr'},'xdspkit'=>{'non_memory_mapped_port'=>'uprev_Shared_BRAM_addr'}}}
  untitled_Shared_BRAM_data_in : xbsIndex_r4/Gateway Out  hdl_port=on  timing_constraint=None  locs_specified=off  LOCs={'B21','B22','A22','B23','B19','C19','A20','A21','A23','B24','A24','A25','E18','D18','C18','B18'}  block_type=gatewayout
      settings: infoedit="Gateway out block.  Converts Xilinx fixed point inputs into ouputs of type Simulink integer, double, or fixed point.<P><P>Hardware notes:  In hardware these blocks become top level output ports or are discarded, depending on how they are configured."  xl_area=[0, 0, 0, 0, 0, 0, 0]  sginterface={'Nallatech'=>{'xdspkit'=>{'non_memory_mapped_port'=>'uprev_Shared_BRAM_data_in'}},'Xilinx'=>{'jtaghwcosim'=>{'non_memory_mapped_port'=>'uprev_Shared_BRAM_data_in'},'xdspkit'=>{'non_memory_mapped_port'=>'uprev_Shared_BRAM_data_in'}}}
  untitled_Shared_BRAM_data_out : xbsIndex_r4/Gateway In  gui_display_data_type=Fixed-point  arith_type=Unsigned  n_bits=32  bin_pt=0  preci_type=Single  exp_width=8  frac_width=24  quantization=Truncate  overflow=Wrap  period=sample_rate  dbl_ovrd=off  timing_constraint=None  locs_specified=off  LOCs={}  hdl_port=on  block_type=gatewayin
      settings: xl_area=[0, 0, 0, 0, 0, 0, 0]
  untitled_Shared_BRAM_we : xbsIndex_r4/Gateway Out  hdl_port=on  timing_constraint=None  locs_specified=off  LOCs={'A14'}  block_type=gatewayout
      settings: infoedit="Gateway out block.  Converts Xilinx fixed point inputs into ouputs of type Simulink integer, double, or fixed point.<P><P>Hardware notes:  In hardware these blocks become top level output ports or are discarded, depending on how they are configured."  xl_area=[0, 0, 0, 0, 0, 0, 0]
  data_out : Outport
  wires:
  munge_in/1(dout) -> convert_din1/1
  munge_out/1(dout) -> data_out/1
  we/1 -> convert_we/1
  addr/1 -> calc_add/1(in)
  mem/1(Out1) -> untitled_Shared_BRAM_data_out/1
  untitled_Shared_BRAM_data_out/1 -> munge_out/1(din)
  convert_we/1 -> untitled_Shared_BRAM_we/1
  untitled_Shared_BRAM_addr/1 -> mem/1(In1)
  untitled_Shared_BRAM_data_in/1 -> mem/2(In2)
  untitled_Shared_BRAM_we/1 -> mem/3(In3)
  calc_add/1(out) -> convert_addr/1
  data_in/1 -> munge_in/1(din)
  convert_din1/1 -> untitled_Shared_BRAM_data_in/1
  convert_addr/1 -> untitled_Shared_BRAM_addr/1
